simulink model "InductionMachineDTC"  (R2026a)
settings: Solver=FixedStepAuto  StopTime=2.5  FixedStep=Ts  MaxStep=1e-3  EnableMultiTasking=on
PreLoadFcn:
  | InductionMachineDTCData;
values from neighbouring files (symbols this model uses):
  fn = 60    [InductionMachineDTCData.m]
  Ki_wr = (wn^2) * (2*H)    (= 218.72)    [InductionMachineDTCData.m]
  Kp_wr = 2 * zeta * wn * (2*H) - F    (= 21.8614)    [InductionMachineDTCData.m]
  p = 2    [InductionMachineDTCData.m]
  psin = (Vn/sqrt(3)*sqrt(2)/wbase)    [InductionMachineDTCData.m]
  Tbase = Pn/(wbase/p)    (= 39.5765291822)    [InductionMachineDTCData.m]    (also in tune_pi.m = Pn/wbase_mech)
  Ts = 5e-6    (= 5e-06)    [InductionMachineDTCData.m]
  Tsc = Ts    (= 5e-06)    [InductionMachineDTCData.m]
  Xls = Lls*Zbase    [InductionMachineDTCData.m]
undefined symbols (not defined in the file or in its folder): ee
libraries: nesl_utility x13, ee_lib x10, fl_lib x9, eeAsmDirectTorqueControl x1, slpidlib x1, simulink x1
Description:
  | Asynchronous Machine Direct Torque Control
settings Model: Creator=The MathWorks, Inc.  LastModifiedBy=rodri
settings DataIOCC: MaxDataPoints=510000  SaveOperatingPoint=on  SaveFormat=StructureWithTime  SignalLoggingName=logsout_InductionMachineDTC
settings DebuggingCC: AlgebraicLoopMsg=error  MultiTaskRateTransMsg=warning
settings HardwareCC: ProdHWDeviceType=32-bit Generic
settings SimscapeCC: SimscapeNominalValues="[{\"value\":\"1\",\"unit\":\"A\"},{\"value\":\"1\",\"unit\":\"bar\"},{\"value\":\"1\",\"unit\":\"cm^2\"},{\"value\":\"1\",\"unit\":\"cm^3/s\"},{\"value\":\"1\",\"unit\":\"kJ/kg\"},{\"value\":\"1\",\"unit\":\"kW\"},{\"value\":\"1\",\"unit\":\"l\"},{\"value\":\"1\",\"unit\":\"N\"},{\"value\":\"1\",\"unit\":\"N*m\"},{\"value\":\"1\",\"unit\":\"V\"}]"  SimscapeLogSimulationStatistics=on  SimscapeLogName=simlog_InductionMachineDTC  SimscapeLogDecimation=5.0  SimscapeLogDataHistory=510000.0

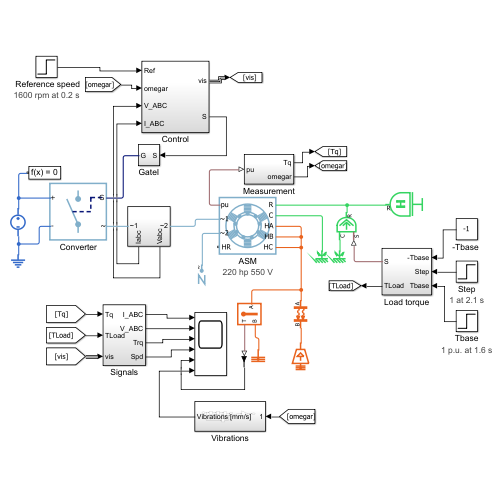
[thumbnail: Simulink's stored preview of the top-level diagram]
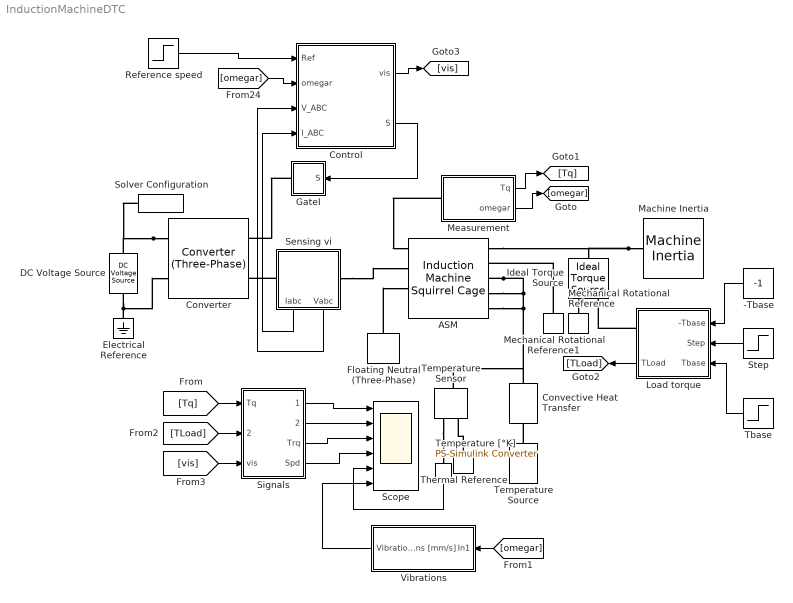
== system InductionMachineDTC ==
  " Reference speed" : Step  Time=0.2  FinalValue=1600  SampleTime=Tsc
      settings: AttributesFormatString=%<After> rpm at %<Time> s
  "-Tbase " : Constant  Value=-1  SampleTime=Ts
  ASM : ee_lib/Electromechanical/Asynchronous/Induction Machine Squirrel Cage  port_option=ee.enum.threePhasePort.composite  SRated=Pn V*A  VRated=Vn V  FRated=fn Hz  nPolePairs=p  param_unit=ee.enum.unit.si  squirrel_cage=ee.enum.squirrelcage.Single  zero_sequence=ee.enum.park.zerosequence.exclude  initialization_option=ee.enum.asm.initialization.fluxvariables  Rs=Rss Ohm  Xls=Xls Ohm  pu_Rs=0.0258  pu_Lls=0.0413  Rrd=Rrr Ohm  Xlrd=Xlr Ohm  pu_Rrd=0.0145  pu_Llrd=0.0424  Rrd1=0.28 Ohm  Xlrd1=0.82 Ohm  Rrd2=0.28 Ohm  Xlrd2=0.82 Ohm  pu_Rrd1=0.0290  pu_Llrd1=0.0848  pu_Rrd2=0.0290  pu_Llrd2=0.0848  Xm=Xm Ohm  pu_Lm=1.7562  X0=Xls Ohm  pu_L0=0.0413  saturation_option=0  saturation_i=[0, 4, 9, 18, 25, 34, 50, 68, 95, 120] A  saturation_v=[0, 88, 154, 198, 220, 242, 264, 286, 308, 330] V  pu_saturation_i=[0, .176, .396, .792, 1.1, 1.496, 2.2, 2.992, 4.18, 5.28]  pu_saturation_v=[0, .4, .7, .9, 1, 1.1, 1.2, 1.3, 1.4, 1.4864]  connection_option=int32(ee.enum.Connection.delta)  angular_position_specify=off  angular_position_priority=None  angular_position=0 deg  angular_position_nominal_specify=off  angular_position_nominal_value=1  angular_position_nominal_unit=deg  pu_psids_specify=off  pu_psids_priority=None  pu_psids=0  pu_psids_nominal_specify=off  pu_psids_nominal_value=1  pu_psids_nominal_unit=1  pu_psiqs_specify=off  pu_psiqs_priority=None  pu_psiqs=0  pu_psiqs_nominal_specify=off  pu_psiqs_nominal_value=1  pu_psiqs_nominal_unit=1  pu_psi0s_specify=off  pu_psi0s_priority=None  pu_psi0s=0  pu_psi0s_nominal_specify=off  pu_psi0s_nominal_value=1  pu_psi0s_nominal_unit=1  pu_psidr_specify=off  pu_psidr_priority=None  pu_psidr=0  pu_psidr_nominal_specify=off  pu_psidr_nominal_value=1  pu_psidr_nominal_unit=1  pu_psiqr_specify=off  pu_psiqr_priority=None  pu_psiqr=0  pu_psiqr_nominal_specify=off  pu_psiqr_nominal_value=1  pu_psiqr_nominal_unit=1  pu_psidr1_specify=off  pu_psidr1_priority=None  pu_psidr1=0  pu_psidr1_nominal_specify=off  pu_psidr1_nominal_value=1  pu_psidr1_nominal_unit=1  pu_psiqr1_specify=off  pu_psiqr1_priority=None  pu_psiqr1=0  pu_psiqr1_nominal_specify=off  pu_psiqr1_nominal_value=1  pu_psiqr1_nominal_unit=1  pu_psidr2_specify=off  pu_psidr2_priority=None  pu_psidr2=0  pu_psidr2_nominal_specify=off  pu_psidr2_nominal_value=1  pu_psidr2_nominal_unit=1  pu_psiqr2_specify=off  pu_psiqr2_priority=None  pu_psiqr2=0  pu_psiqr2_nominal_specify=off  pu_psiqr2_nominal_value=1  pu_psiqr2_nominal_unit=1  psids_specify=off  psids_priority=None  psids=0 Wb  psids_nominal_specify=off  psids_nominal_value=1  psids_nominal_unit=Wb  psiqs_specify=off  psiqs_priority=None  psiqs=0 Wb  psiqs_nominal_specify=off  psiqs_nominal_value=1  psiqs_nominal_unit=Wb  psi0s_specify=off  psi0s_priority=None  psi0s=0 Wb  psi0s_nominal_specify=off  psi0s_nominal_value=1  psi0s_nominal_unit=Wb  psidr_specify=off  psidr_priority=None  psidr=0 Wb  psidr_nominal_specify=off  psidr_nominal_value=1  psidr_nominal_unit=Wb  psiqr_specify=off  psiqr_priority=None  psiqr=0 Wb  psiqr_nominal_specify=off  psiqr_nominal_value=1  psiqr_nominal_unit=Wb  psidr1_specify=off  psidr1_priority=None  psidr1=0 Wb  psidr1_nominal_specify=off  psidr1_nominal_value=1  psidr1_nominal_unit=Wb  psiqr1_specify=off  psiqr1_priority=None  psiqr1=0 Wb  psiqr1_nominal_specify=off  psiqr1_nominal_value=1  psiqr1_nominal_unit=Wb  psidr2_specify=off  psidr2_priority=None  psidr2=0 Wb  psidr2_nominal_specify=off  psidr2_nominal_value=1  psidr2_nominal_unit=Wb  psiqr2_specify=off  psiqr2_priority=None  psiqr2=0 Wb  psiqr2_nominal_specify=off  psiqr2_nominal_value=1  psiqr2_nominal_unit=Wb  slip_specify=off  slip_priority=None  slip=0  slip_nominal_specify=off  slip_nominal_value=1  slip_nominal_unit=1  real_power_generated_specify=off  real_power_generated_priority=None  real_power_generated=0 W  real_power_generated_nominal_specify=off  real_power_generated_nominal_value=1  real_power_generated_nominal_unit=W  mechanical_power_consumed_specify=off  mechanical_power_consumed_priority=None  mechanical_power_consumed=0 W  mechanical_power_consumed_nominal_specify=off  mechanical_power_consumed_nominal_value=1  mechanical_power_consumed_nominal_unit=W  Tmeas=298.15 K  alpha=3.93e-3 1/K  alpha_cage=4.4e-3 1/K  stator_thermal_mass=100 J/K  rotor_thermal_mass=200 J/K  temperatureA_specify=off  temperatureA_priority=High  temperatureA=25 degC  temperatureA_nominal_specify=off  temperatureA_nominal_value=1  temperatureA_nominal_unit=degC  temperatureB_specify=off  temperatureB_priority=High  temperatureB=25 degC  temperatureB_nominal_specify=off  temperatureB_nominal_value=1  temperatureB_nominal_unit=degC  temperatureC_specify=off  temperatureC_priority=High  temperatureC=25 degC  temperatureC_nominal_specify=off  temperatureC_nominal_value=1  temperatureC_nominal_unit=degC  temperatureR_specify=off  temperatureR_priority=High  temperatureR=25 degC  temperatureR_nominal_specify=off  temperatureR_nominal_value=1  temperatureR_nominal_unit=degC
      settings: AttributesFormatString=220 hp 550 V
  Control : Subsystem
  Convective Heat Transfer : fl_lib/Thermal/Thermal Elements/Convective Heat Transfer  thermal_type=foundation.enum.constant_variable.constant  area=1e-4 m^2  heat_tr_coeff=20 W/(K*m^2)  min_heat_tr_coeff=1e-3 W/(K*m^2)  T_specify=off  T_priority=None  T=0 K  T_nominal_specify=off  T_nominal_value=1  T_nominal_unit=K  Q_specify=off  Q_priority=None  Q=0 W  Q_nominal_specify=off  Q_nominal_value=1  Q_nominal_unit=W
  Converter : ee_lib/Semiconductors & Converters/Converters/Converter (Three-Phase)  port_option=ee.enum.threePhasePort.composite  fidelity_option=ee.enum.converters.fidelity.detailed  device_type=3  showThermalPort=false  K=0  Vth=0.5 V  Vgt=1 V  Vgt_off=-1 V  Ih=1 A  Vf=0.8 V  Ron=0.001 Ohm  Rds=0.001 Ohm  Goff=1e-5 1/Ohm  Eon_scalar=22.86e-3 J  Eoff_scalar=17.14e-3 J  Eoff_natural_commutation=10e-3 J  Voff=300 V  Iout_scalar=600 A  onCurrentMeasDelay=0 s  useCurrentFromPreviousCycle=false  useVoltageFromPreviousCycle=false  diode_param=2  diode_Vf=0.8 V  diode_Ron=0.001 Ohm  diode_Goff=1e-5 1/Ohm  diode_C=50 nF  diode_iRM=-235 A  diode_iF=300 A  diode_idot=-50 A/us  diode_trr_param=1  diode_trr_factor=3  diode_trr=15 us  diode_Qrr=1.5e+3 s*uA  diode_rec_loss_model=ee.enum.diode.reverseRecoveryModel.fixed  diode_ErecVal=0 J  diode_scaleWithIandV=false  diode_ErecMat=zeros(2, 3) J  diode_TjrecVec=[298.15, 398.15] K  diode_IfrecVec=[.1, 1, 10] A  diode_IrecVal=10 A  diode_VrecVal=10 V  diode_tFilter=1 / 1000 / 100 s  thermal_network_parameterization=ee.enum.thermalNetworkTopology.external  Rth=[.08, .5] K/W  Rth_Cauer=[.08, .1, .5] K/W  Rth_Foster=[.08, .14, .22, .16] K/W  thermal_mass_parameterization=ee.enum.thermalNetwork.timeconstant  thermal_mass=[.01, .5] J/K  thermal_mass_Cauer=[.01, .1, .5] J/K  thermal_mass_Foster=[.001, .005, .05, .5] J/K  thermal_time_constant=[.001, .2] s  thermal_time_constant_Cauer=[.001, .1, .2] s  thermal_time_constant_Foster=[7e-05, .0007, .01, .08] s  thermal_mass_initial_temperatures=[25, 25] degC  thermal_mass_initial_temperatures_Cauer=[25, 25, 25] degC  junction_thermal_mass=0.01 J/K  Tvec_initial_Foster=[25, 25, 25, 25] degC  snubber_type=0  Cs=1e-7 F  Rs=0.1 Ohm  Vce_loss=[0, 150, 300] V
  DC Voltage Source : fl_lib/Electrical/Electrical Sources/DC Voltage Source  v0=750 V
  Electrical Reference : fl_lib/Electrical/Electrical Elements/Electrical Reference
  Floating Neutral (Three-Phase) : ee_lib/Connectors & References/Floating Neutral (Three-Phase)  port_option=ee.enum.threePhasePort.composite  G_parasitic=1e-6 1/Ohm
  GateI : Subsystem
  Ideal Torque Source : fl_lib/Mechanical/Mechanical Sources/Ideal Torque Source
  Load torque : Subsystem
      settings: PortSchema="{\"entries\":[{\"content\":{\"sides\":[{\"content\":{\"connectorIds\":[\"In1\",\"In2\",\"In3\"]},\"type\":\"ConnectorPlacement.EquallySpacedRectSide\",\"uuid\":\"c233883d-7645-4c8d-bbcf-02207cfb42e0\"},{\"content\":{\"connectorIds\":[\"RConn1\",\"Out1\"],\"side\":\"RIGHT\"},\"type\":\"ConnectorPlacement.EquallySpacedRectSide\",\"uuid\":\"2628e6dc-936a-4322-ae7b-8d160878f868\"},{\"content\":{\"connectorIds\":[],\"side\":\"TOP\"},\"type\":\"ConnectorPlacement.EquallySpacedRectSide\",\"uuid\":\"80e56048-a4aa-4d37-84cc-2dd4e039608f\"}]},\"type\":\"ConnectorPlacement.EquallySpacedConnector\",\"uuid\":\"37ec6042-3a1f-4092-a886-8852041d841b\"}],\"packageUris\":[\"http://schema.mathworks.com/mf0/Connector/R2020b\"],\"version\":\"1.0\"}"
  Machine Inertia : ee_lib/Electromechanical/Mechanical/Machine Inertia  SRated=Pn V*A  FRated=fn Hz  nPolePairs=p  inertia_option=2  J=0.1148 kg*m^2  H=H s*W/V/A  damper_option=2  D=0.00222 N*m/(rad/s)  pu_D=F  initialization_option=2  fMechanical0=60 Hz  fElectrical0=0 Hz
  Measurement : Subsystem
      settings: PortSchema="{\"entries\":[{\"content\":{\"sides\":[{\"content\":{\"connectorIds\":[\"Out1\",\"Out2\"]},\"type\":\"ConnectorPlacement.EquallySpacedRectSide\",\"uuid\":\"bc88329e-50f2-4c79-b51c-8554cd6cb4a7\"},{\"content\":{\"connectorIds\":[\"RConn1\"],\"side\":\"RIGHT\"},\"type\":\"ConnectorPlacement.EquallySpacedRectSide\",\"uuid\":\"4ae5b1ab-fe56-4c08-abcc-052ba619d9b7\"},{\"content\":{\"side\":\"TOP\"},\"type\":\"ConnectorPlacement.EquallySpacedRectSide\",\"uuid\":\"4a72e2c5-964f-4562-8af1-645c6fe3acb6\"}]},\"type\":\"ConnectorPlacement.EquallySpacedConnector\",\"uuid\":\"fc44c596-f6a7-440e-ae04-cb8373d14ea8\"}],\"packageUris\":[\"http://schema.mathworks.com/mf0/Connector/R2020b\"],\"version\":\"1.0\"}"
  Mechanical Rotational Reference : fl_lib/Mechanical/Rotational Elements/Mechanical Rotational Reference
  Mechanical Rotational Reference1 : fl_lib/Mechanical/Rotational Elements/Mechanical Rotational Reference
  Scope : Scope  NumInputPorts=6
      settings: ActiveDisplayYMinimum=-106.27621516175316  ActiveDisplayYMaximum=101.30997487488192
  Sensing vi : Subsystem
      settings: PortSchema="{\"entries\":[{\"content\":{\"sides\":[{\"content\":{\"connectorIds\":[\"LConn1\"]},\"type\":\"ConnectorPlacement.EquallySpacedRectSide\",\"uuid\":\"c5057f2e-2c18-4118-b873-a75143a124e4\"},{\"content\":{\"connectorIds\":[\"RConn1\"],\"side\":\"RIGHT\"},\"type\":\"ConnectorPlacement.EquallySpacedRectSide\",\"uuid\":\"847dbac9-66f5-462a-b095-b42c8738b9ce\"},{\"content\":{\"connectorIds\":[],\"side\":\"TOP\"},\"type\":\"ConnectorPlacement.EquallySpacedRectSide\",\"uuid\":\"1cd52aa7-c39c-45ef-b799-a348546c5bc9\"},{\"content\":{\"connectorIds\":[\"Out1\",\"Out2\"],\"side\":\"BOTTOM\"},\"type\":\"ConnectorPlacement.EquallySpacedRectSide\",\"uuid\":\"68147b4d-d600-401c-916d-5bcceac84bb7\"}]},\"type\":\"ConnectorPlacement.EquallySpacedConnector\",\"uuid\":\"7d89bf63-b784-4419-8d3e-10ce7abb2518\"}],\"packageUris\":[\"http://schema.mathworks.com/mf0/Connector/R2020b\"],\"version\":\"1.0\"}"
  Signals : Subsystem
  Solver Configuration : nesl_utility/Solver Configuration  PhysicalDomain=network_engine_domain  SubClassName=solver  LeftPortType=input  RightPortType=generic  Tones=[]  Harmonics=[]  SimulateNoise=off  Profile=off  UseLocalSampling=off  EnableSwitchedLinearOptims=on  FrequencyDomain=off  UseCCode=off  RelTol=0.001  AbsTol=1e-06  MinStep=1e-09  ToWorkspace=off  RevertToSquareIcSolve=off  NumHomotopyIterations=100  PhasorMode=off  PhasorModeNumHarmonics=1  ConsistencySolver=NEWTON_FTOL  CanonicalOrdering=UNORDERED  OptimizeIntermediates=UNOPTIMIZED  IndexReductionMethod=DerivativeReplacement  DoDC=off  ResidualTolerance=1e-09  ConsistencyTolSource=GLOBAL  ConsistencyAbsTol=0.001  ConsistencyRelTol=0.001  ConsistencyTolFactor=0.001  UseLocalSolver=on  LocalSolverChoice=NE_BACKWARD_EULER_ADVANCER  ResolveIndetEquations=on  FunctionEvalNumThread=1  LocalSolverSampleTime=Ts  DoFixedCost=on  MaxNonlinIter=5  MaxModeIter=2  ComputeImpulses=off  ImpulseIterations=2  LinearAlgebra=auto  LinearAlgebraNumThread=0  EquationFormulation=NE_TIME_EF  DelaysMemoryBudget=1024  AutomaticFiltering=on  FilteringTimeConstant=0.001  PartitionStorageMethod=AS_NEEDED  PartitionMemoryBudget=1024  PartitionMethod=ROBUST  MultibodyUseLocalSolver=off  MultibodyLocalSolverChoice=ODE1  MultibodyLocalSolverSampleTime=0.001
  Step : Step  Time=2.1  SampleTime=Ts
      settings: AttributesFormatString=%<After> at %<Time> s
  Tbase : Step  Time=1.6  SampleTime=Ts
      settings: AttributesFormatString=%<After> p.u. at %<Time> s
  Temperature Sensor : fl_lib/Thermal/Thermal Sensors/Temperature Sensor  temperature_measure=foundation.enum.MeasurementReference.difference
  Temperature Source : fl_lib/Thermal/Thermal Sources/Temperature Source  temperature=298.15 K
  Temperature [°K] : nesl_utility/PS-Simulink Converter  PhysicalDomain=network_engine_domain  SubClassName=ps_output  LeftPortType=input  RightPortType=output  PseudoPeriodic=off  Frequencies=[]  VectorFormat=inherit  Unit=inherit  AffineConversion=off
  Thermal Reference : fl_lib/Thermal/Thermal Elements/Thermal Reference
  Vibrations : Subsystem
  wires:
  Temperature [°K]/1 -> Scope/5
  Step/1 -> Load torque/2(Step)
  Measurement/1(Tq) -> [Tq]
  [omegar] -> Control/2(omegar)
  Signals/4(Spd) -> Scope/4
  " Reference speed"/1 -> Control/1(Ref)
  Load torque/1(TLoad) -> [TLoad]
  Control/1(vis) -> [vis]
  "-Tbase "/1 -> Load torque/1(-Tbase)
  Control/2(S) -> GateI/1(S)
  [TLoad] -> Signals/2(TLoad)
  Measurement/2(omegar) -> [omegar]
  Sensing vi/1(Iabc) -> Control/4(I_ABC)
  Signals/1(I_ABC) -> Scope/1
  Sensing vi/2(Vabc) -> Control/3(V_ABC)
  Tbase/1 -> Load torque/3(Tbase)
  Signals/3(Trq) -> Scope/3
  Signals/2(V_ABC) -> Scope/2
  [Tq] -> Signals/1(Tq)
  [vis] -> Signals/3(vis)
  [omegar] -> Vibrations/1(In1)
  Vibrations/1(Vibrations [mm/s]) -> Scope/6
  connections:
  DC Voltage Source/RConn1 -- Electrical Reference/LConn1 -- Converter/RConn2
  ASM/LConn3 -- ASM/LConn4 -- Temperature Sensor/LConn1 -- Convective Heat Transfer/LConn1 -- ASM/LConn5
  Converter/RConn1 -- DC Voltage Source/LConn1 -- Solver Configuration/RConn1
  Machine Inertia/LConn1 -- Ideal Torque Source/LConn1 -- ASM/LConn1
  Temperature Source/LConn1 -- Convective Heat Transfer/RConn1
  Mechanical Rotational Reference1/LConn1 -- ASM/LConn2
  Load torque/RConn1 -- Ideal Torque Source/RConn1
  Thermal Reference/LConn1 -- Temperature Sensor/RConn1
  Measurement/RConn1 -- ASM/RConn1
  Sensing vi/LConn1 -- Converter/LConn2
  GateI/RConn1 -- Converter/LConn1
  Temperature Sensor/RConn2 -- Temperature [°K]/LConn1
  Floating Neutral (Three-Phase)/LConn1 -- ASM/RConn3
  Ideal Torque Source/RConn2 -- Mechanical Rotational Reference/LConn1
  Sensing vi/RConn1 -- ASM/RConn2

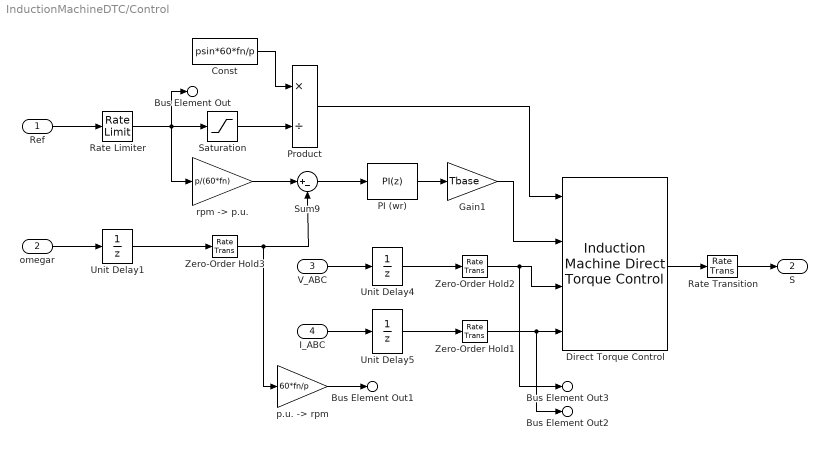
== system InductionMachineDTC/Control ==
  Ref : Inport
  omegar : Inport  Port=2
  V_ABC : Inport  Port=3
  I_ABC : Inport  Port=4
  " Direct Torque Control" : eeAsmDirectTorqueControl/Induction Machine Direct Torque Control  Rs=Rss  p=p  FluxHystBand=FluxHystBand  THystBand=THystBand  Ts=Tsc
  Const : Constant  Value=psin*60*fn/p
  Gain1 : Gain  Gain=Tbase
  PI (wr) : slpidlib/PID Controller  Controller=PI  Form=Parallel  TimeDomain=Discrete-time  UseExternalTs=off  SampleTime=Tsc  IntegratorMethod=Forward Euler  FilterMethod=Forward Euler  ControllerParametersSource=internal  P=Kp_wr  I=Ki_wr  UseKiTs=off  D=0  UseExternalDerivativeSource=off  N=100  UseFilter=on  TunerSelectOption=Transfer Function Based (PID Tuner App)  InitialConditionSource=internal  InitialConditionForIntegrator=0  InitialConditionForFilter=0  DifferentiatorICPrevScaledInput=0  ExternalReset=none  TrackingMode=off  Kt=1  LimitOutput=on  SatLimitsSource=internal  UpperSaturationLimit=2  LowerSaturationLimit=-2  LinearizeAsGain=on  AntiWindupMode=back-calculation  Kb=1000  LimitIntegrator=off  UpperIntegratorSaturationLimit=inf  LowerIntegratorSaturationLimit=-inf  POutMin=[]  POutMax=[]  IOutMin=[]  IOutMax=[]  DOutMin=[]  DOutMax=[]  NOutMin=[]  NOutMax=[]  SumOutMin=[]  SumOutMax=[]  SaturationOutMin=[]  SaturationOutMax=[]  PParamMin=[]  PParamMax=[]  IParamMin=[]  IParamMax=[]  DParamMin=[]  DParamMax=[]  NParamMin=[]  NParamMax=[]  KbParamMin=[]  KbParamMax=[]  KtParamMin=[]  KtParamMax=[]  KbOutMin=[]  KbOutMax=[]  KtOutMin=[]  KtOutMax=[]  IntegratorOutMin=[]  IntegratorOutMax=[]  FilterOutMin=[]  FilterOutMax=[]  SumI1OutMin=[]  SumI1OutMax=[]  SumI2OutMin=[]  SumI2OutMax=[]  SumI3OutMin=[]  SumI3OutMax=[]  SumI4OutMin=[]  SumI4OutMax=[]  SumDOutMin=[]  SumDOutMax=[]  DifferentiatorOutMin=[]  DifferentiatorOutMax=[]  FilterDiffOutCoefMin=[]  FilterDiffOutCoefMax=[]  ReciprocalOutMin=[]  ReciprocalOutMax=[]  SumDenOutMin=[]  SumDenOutMax=[]  SumNumOutMin=[]  SumNumOutMax=[]  DivideOutMin=[]  DivideOutMax=[]  UdiffTsProdOutMin=[]  UdiffTsProdOutMax=[]  NTsProdOutMin=[]  NTsProdOutMax=[]  UintegralTsProdOutMin=[]  UintegralTsProdOutMax=[]  UngainTsProdOutMin=[]  UngainTsProdOutMax=[]  ClampingZeroOutDataTypeStr=Inherit: Inherit via back propagation  ClampingZeroOutMin=[]  ClampingZeroOutMax=[]  FilterDenConstantOutDataTypeStr=Inherit: Inherit via back propagation  FilterDenConstantOutMin=[]  FilterDenConstantOutMax=[]  PCopyOutDataTypeStr=Inherit: Inherit via back propagation  PCopyOutMin=[]  PCopyOutMax=[]  NCopyOutDataTypeStr=Inherit: Inherit via back propagation  NCopyOutMin=[]  NCopyOutMax=[]  IntegratorContinuousStateAttributes=''  IntegratorStateMustResolveToSignalObject=off  IntegratorRTWStateStorageClass=Auto  FilterContinuousStateAttributes=''  FilterStateMustResolveToSignalObject=off  FilterRTWStateStorageClass=Auto  ParallelPVariant=InternalParameters  IdealPVariant=Disabled  IVariant=InternalParameters  DVariant=Disabled  IntegratorVariant=Discrete  SatVariant=Enabled  AWVariant=BackCalculation  PCopyVariant=Disabled  TRVariant=Disabled  FdbkBlocksVariant=Forward  IdealPFdbkVariant=Disabled  SatFdbkVariant=Disabled  DerivativeFilterVariant=Disabled  NVariant=Disabled  NCopyVariant=Disabled_SignalSpec  FilterICVariant=Disabled  IntegratorICVariant=InternalICs  ExternalResetVariant=Disabled  TRSumVariant=Passthrough  SumFdbkVariant=Disabled  SumVariant=Sum_PI  TsampFilterVariant=InternalTs  TsampNgainVariant=Passthrough  TsampIntegralVariant=Disabled_SignalSpec  ExternalSaturationOutDataTypeStr=Inherit: Same as second input  DerivativeSourceVariant=Disabled  PreIntVariant=InternalPreInt
  Product : Product  Inputs=*/
  Rate Limiter : RateLimiter  RisingSlewLimit=2000  FallingSlewLimit=-2000  SampleTimeMode=inherited
      settings: AttributesFormatString=%<RisingSlewLimit> rpm/s
  Rate Transition : RateTransition
  Saturation : Saturate  UpperLimit=inf  LowerLimit=60*fn/p
  Sum9 : Sum  Inputs=|+-
  Unit Delay1 : UnitDelay  SampleTime=Ts
  Unit Delay4 : UnitDelay  SampleTime=Ts
  Unit Delay5 : UnitDelay  SampleTime=Ts
  Zero-Order Hold1 : RateTransition
  Zero-Order Hold2 : RateTransition
  Zero-Order Hold3 : RateTransition
  "p.u. -> rpm" : Gain  Gain=60*fn/p
  "rpm -> p.u." : Gain  Gain=p/(60*fn)
  Bus Element Out : Outport  PortName=vis  Element=SpdRef
  Bus Element Out1 : Outport  PortName=vis  Element=Spd
  Bus Element Out2 : Outport  PortName=vis  Element=Iabc
  Bus Element Out3 : Outport  PortName=vis  Element=Vabc
  S : Outport  Port=2  VectorParamsAs1DForOutWhenUnconnected=off
  wires:
  Ref/1 -> Rate Limiter/1
  omegar/1 -> Unit Delay1/1
  Saturation/1 -> Product/2
  Zero-Order Hold3/1 -> "p.u. -> rpm"/1, Sum9/2
  Const/1 -> Product/1
  Unit Delay1/1 -> Zero-Order Hold3/1
  Rate Limiter/1 -> "rpm -> p.u."/1, Saturation/1, Bus Element Out/1
  "rpm -> p.u."/1 -> Sum9/1
  Product/1 -> " Direct Torque Control"/1
  Sum9/1 -> PI (wr)/1
  Rate Transition/1 -> S/1
  V_ABC/1 -> Unit Delay4/1
  I_ABC/1 -> Unit Delay5/1
  "p.u. -> rpm"/1 -> Bus Element Out1/1
  PI (wr)/1 -> Gain1/1
  Unit Delay4/1 -> Zero-Order Hold2/1
  Unit Delay5/1 -> Zero-Order Hold1/1
  Gain1/1 -> " Direct Torque Control"/2
  Zero-Order Hold2/1 -> " Direct Torque Control"/3, Bus Element Out3/1
  Zero-Order Hold1/1 -> " Direct Torque Control"/4, Bus Element Out2/1
  " Direct Torque Control"/1 -> Rate Transition/1

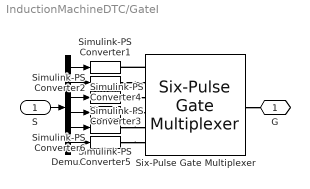
== system InductionMachineDTC/GateI ==
  S : Inport
  Demux : Demux  Outputs=6
  Simulink-PS Converter{1..6} (6 alike) : nesl_utility/Simulink-PS Converter  PhysicalDomain=network_engine_domain  SubClassName=ps_input  LeftPortType=input  RightPortType=output  PseudoPeriodic=off  Frequencies=[]  NoiseDistribution=none  NoiseParameters=[]  Unit=1  AffineConversion=off  FilteringAndDerivatives=zero  SimscapeFilterOrder=1  InputFilterTimeConstant=0.001  UdotUserProvided=1
  Six-Pulse Gate Multiplexer : ee_lib/Semiconductors & Converters/Converters/Six-Pulse Gate Multiplexer  port_option=ee.enum.controlport.ps
  G : PMIOPort  Side=Right
  wires:
  Demux/3 -> Simulink-PS Converter3/1
  Demux/6 -> Simulink-PS Converter6/1
  Demux/5 -> Simulink-PS Converter5/1
  S/1 -> Demux/1
  Demux/2 -> Simulink-PS Converter2/1
  Demux/1 -> Simulink-PS Converter1/1
  Demux/4 -> Simulink-PS Converter4/1
  connections:
  Six-Pulse Gate Multiplexer/RConn1 -- G/RConn1
  Six-Pulse Gate Multiplexer/LConn1 -- Simulink-PS Converter1/RConn1
  Simulink-PS Converter5/RConn1 -- Six-Pulse Gate Multiplexer/LConn5
  Simulink-PS Converter6/RConn1 -- Six-Pulse Gate Multiplexer/LConn6
  Simulink-PS Converter3/RConn1 -- Six-Pulse Gate Multiplexer/LConn3
  Simulink-PS Converter2/RConn1 -- Six-Pulse Gate Multiplexer/LConn2
  Simulink-PS Converter4/RConn1 -- Six-Pulse Gate Multiplexer/LConn4

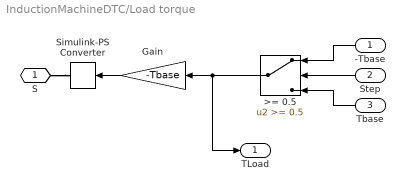
== system InductionMachineDTC/Load torque ==
  -Tbase : Inport
  Step : Inport  Port=2
  Tbase : Inport  Port=3
  ">= 0.5 " : Switch  Threshold=0.5  SaturateOnIntegerOverflow=off  InputSameDT=off
  Gain : Gain  Gain=-Tbase
  Simulink-PS Converter : nesl_utility/Simulink-PS Converter  PhysicalDomain=network_engine_domain  SubClassName=ps_input  LeftPortType=input  RightPortType=output  PseudoPeriodic=off  Frequencies=[]  NoiseDistribution=none  NoiseParameters=[]  Unit=1  AffineConversion=off  FilteringAndDerivatives=zero  SimscapeFilterOrder=1  InputFilterTimeConstant=0.001  UdotUserProvided=1
  S : PMIOPort  Side=Right
  TLoad : Outport
  wires:
  Gain/1 -> Simulink-PS Converter/1
  ">= 0.5 "/1 -> TLoad/1, Gain/1
  -Tbase/1 -> ">= 0.5 "/1
  Step/1 -> ">= 0.5 "/2
  Tbase/1 -> ">= 0.5 "/3
  connections:
  S/RConn1 -- Simulink-PS Converter/RConn1

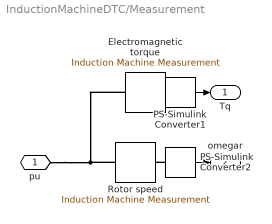
== system InductionMachineDTC/Measurement ==
  Electromagnetic torque : ee_lib/Electromechanical/Asynchronous/Induction Machine Measurement  output_idx=1
  PS-Simulink Converter1 : nesl_utility/PS-Simulink Converter  PhysicalDomain=network_engine_domain  SubClassName=ps_output  LeftPortType=input  RightPortType=output  PseudoPeriodic=off  Frequencies=[]  VectorFormat=1-D array  Unit=1  AffineConversion=off
  PS-Simulink Converter2 : nesl_utility/PS-Simulink Converter  PhysicalDomain=network_engine_domain  SubClassName=ps_output  LeftPortType=input  RightPortType=output  PseudoPeriodic=off  Frequencies=[]  VectorFormat=1-D array  Unit=1  AffineConversion=off
  Rotor speed : ee_lib/Electromechanical/Asynchronous/Induction Machine Measurement  output_idx=2
  pu : PMIOPort  Side=Right
  Tq : Outport
  omegar : Outport  Port=2
  wires:
  PS-Simulink Converter2/1 -> omegar/1
  PS-Simulink Converter1/1 -> Tq/1
  connections:
  PS-Simulink Converter2/LConn1 -- Rotor speed/RConn1
  PS-Simulink Converter1/LConn1 -- Electromagnetic torque/RConn1
  Electromagnetic torque/LConn1 -- pu/RConn1 -- Rotor speed/LConn1

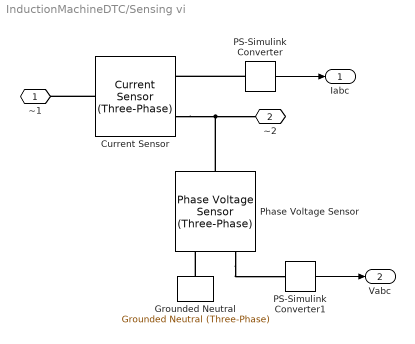
== system InductionMachineDTC/Sensing vi ==
  Current Sensor : ee_lib/Sensors & Transducers/Current Sensor (Three-Phase)  port_option=ee.enum.threePhasePort.composite
  Grounded Neutral : ee_lib/Connectors & References/Grounded Neutral (Three-Phase)  port_option=ee.enum.threePhasePort.composite
  PS-Simulink Converter : nesl_utility/PS-Simulink Converter  PhysicalDomain=network_engine_domain  SubClassName=ps_output  LeftPortType=input  RightPortType=output  PseudoPeriodic=off  Frequencies=[]  VectorFormat=1-D array  Unit=A  AffineConversion=off
  PS-Simulink Converter1 : nesl_utility/PS-Simulink Converter  PhysicalDomain=network_engine_domain  SubClassName=ps_output  LeftPortType=input  RightPortType=output  PseudoPeriodic=off  Frequencies=[]  VectorFormat=1-D array  Unit=V  AffineConversion=off
  Phase Voltage Sensor : ee_lib/Sensors & Transducers/Phase Voltage Sensor (Three-Phase)  port_option=ee.enum.threePhasePort.composite
  ~1 : PMIOPort  Side=Left
  ~2 : PMIOPort  Port=2  Side=Right
  Iabc : Outport
  Vabc : Outport  Port=2
  wires:
  PS-Simulink Converter/1 -> Iabc/1
  PS-Simulink Converter1/1 -> Vabc/1
  connections:
  Current Sensor/LConn1 -- ~1/RConn1
  PS-Simulink Converter/LConn1 -- Current Sensor/RConn1
  Current Sensor/RConn2 -- Phase Voltage Sensor/LConn1 -- ~2/RConn1
  Phase Voltage Sensor/RConn1 -- PS-Simulink Converter1/LConn1
  Grounded Neutral/LConn1 -- Phase Voltage Sensor/RConn2

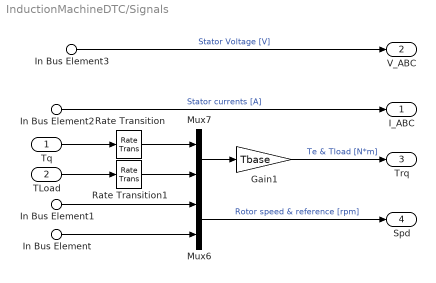
== system InductionMachineDTC/Signals ==
  Tq : Inport
  TLoad : Inport  Port=2
  In Bus Element : Inport  Port=3  PortName=vis  Element=SpdRef
  In Bus Element1 : Inport  Port=3  PortName=vis  Element=Spd
  In Bus Element2 : Inport  Port=3  PortName=vis  Element=Iabc
  In Bus Element3 : Inport  Port=3  PortName=vis  Element=Vabc
  Gain1 : Gain  Gain=Tbase
  Mux6 : Mux  Inputs=2
  Mux7 : Mux  Inputs=2
  Rate Transition : RateTransition
  Rate Transition1 : RateTransition
  I_ABC : Outport  VectorParamsAs1DForOutWhenUnconnected=off
  V_ABC : Outport  Port=2
  Trq : Outport  Port=3  VectorParamsAs1DForOutWhenUnconnected=off
  Spd : Outport  Port=4  VectorParamsAs1DForOutWhenUnconnected=off
  wires:
  In Bus Element2/1 -> I_ABC/1  "Stator currents [A]"
  Mux7/1 -> Gain1/1
  Tq/1 -> Rate Transition/1
  In Bus Element/1 -> Mux6/2
  Mux6/1 -> Spd/1  "Rotor speed & reference [rpm]"
  TLoad/1 -> Rate Transition1/1
  Gain1/1 -> Trq/1  "Te & Tload [N*m]"
  In Bus Element1/1 -> Mux6/1
  Rate Transition/1 -> Mux7/1
  Rate Transition1/1 -> Mux7/2
  In Bus Element3/1 -> V_ABC/1  "Stator Voltage [V]"

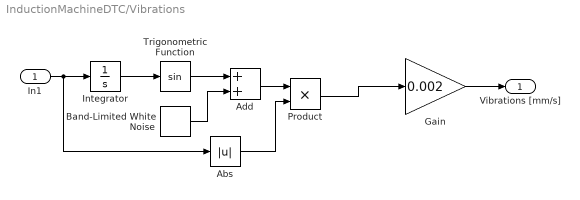
== system InductionMachineDTC/Vibrations ==
  In1 : Inport
  Abs : Abs  SaturateOnIntegerOverflow=off
  Add : Sum
  Band-Limited White Noise : simulink/Sources/Band-Limited White Noise  Cov=[0.1]  Ts=Ts  seed=[23341]
  Gain : Gain  Gain=0.002
  Integrator : Integrator
  Product : Product
  Trigonometric Function : Trigonometry  OutputSignalType=real
  Vibrations [mm/s] : Outport
  wires:
  In1/1 -> Abs/1, Integrator/1
  Integrator/1 -> Trigonometric Function/1
  Band-Limited White Noise/1 -> Add/2
  Trigonometric Function/1 -> Add/1
  Gain/1 -> Vibrations [mm/s]/1
  Add/1 -> Product/1
  Abs/1 -> Product/2
  Product/1 -> Gain/1
